simulink model "Robot"  (R2026a)
settings: Solver=ode1  StopTime=30  FixedStep=2e-5
model workspace (MAT data in the model file):
  bt_seed = 0
  pose0 = [0; 0; 0]
  theta_seed = 0
  x_seed = 0
  y_seed = 0
values from neighbouring files (symbols this model uses):
  bias_th = 0.000    (= 0)    [run_simulation.m]
  bias_x = 0.000    (= 0)    [run_simulation.m]
  bias_y = 0.000    (= 0)    [run_simulation.m]
  CAM_LAT = 0.08    [run_simulation.m]
  L_track = 0.136    [run_simulation.m]
  R_wheel = 0.065/2    (= 0.0325)    [run_simulation.m]
  sig_th = 0.035    [run_simulation.m]
  sig_xy = 0.002    [run_simulation.m]
  Ts_cam = 1/25    (= 0.04)    [run_simulation.m]
settings Model: ParameterArgumentNames=bt_seed,pose0,theta_seed,x_seed,y_seed  Creator=AdrianStark  LastModifiedBy=AdrianStark
settings ModelReferenceCC: ModelReferenceMinAlgLoopOccurrences=on

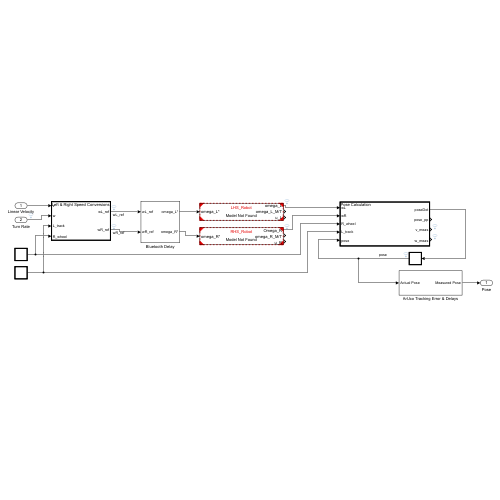
[thumbnail: Simulink's stored preview of the top-level diagram]
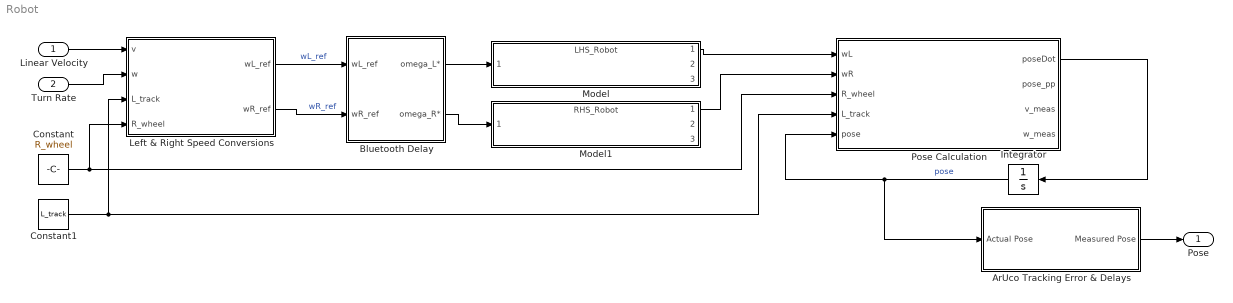
== system Robot ==
  Linear Velocity : Inport
  Turn Rate : Inport  Port=2
  ArUco Tracking Error & Delays : Subsystem
  Bluetooth Delay : Subsystem
  Constant : Constant  Value=R_wheel
  Constant1 : Constant  Value=L_track
  Integrator : Integrator  InitialCondition=pose0
  Left & Right Speed Conversions : MATLAB Function  TreatAsAtomicUnit=on
  Model : ModelReference  ModelNameDialog=LHS_Robot  SimulationMode=Normal  ModelReferenceVersion=1.40
  Model1 : ModelReference  ModelNameDialog=RHS_Robot  SimulationMode=Normal  ModelReferenceVersion=1.40
  Pose Calculation : MATLAB Function  TreatAsAtomicUnit=on
  Pose : Outport
  wires:
  Linear Velocity/1 -> Left & Right Speed Conversions/1(v)
  Turn Rate/1 -> Left & Right Speed Conversions/2(w)
  Pose Calculation/1(poseDot) -> Integrator/1
  Integrator/1 -> ArUco Tracking Error & Delays/1(Actual Pose), Pose Calculation/5(pose)  "pose"
  Constant/1 -> Left & Right Speed Conversions/4(R_wheel), Pose Calculation/3(R_wheel)
  Constant1/1 -> Left & Right Speed Conversions/3(L_track), Pose Calculation/4(L_track)
  Bluetooth Delay/1(omega_L*) -> Model/1
  Bluetooth Delay/2(omega_R*) -> Model1/1
  Left & Right Speed Conversions/2(wR_ref) -> Bluetooth Delay/2(wR_ref)  "wR_ref"
  Left & Right Speed Conversions/1(wL_ref) -> Bluetooth Delay/1(wL_ref)  "wL_ref"
  ArUco Tracking Error & Delays/1(Measured Pose) -> Pose/1
  Model1/1 -> Pose Calculation/2(wR)
  Model/1 -> Pose Calculation/1(wL)

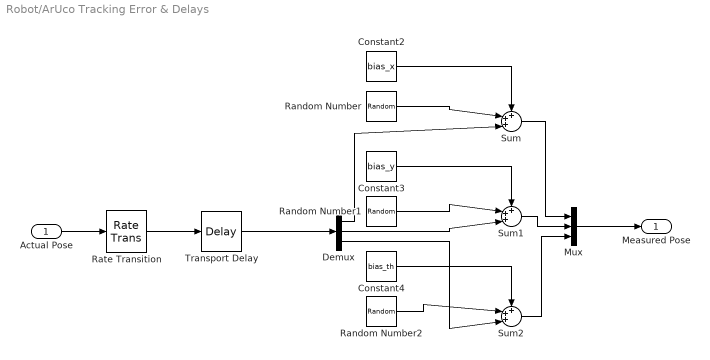
== system Robot/ArUco Tracking Error & Delays ==
  Actual Pose : Inport
  Constant2 : Constant  Value=bias_x
  Constant3 : Constant  Value=bias_y
  Constant4 : Constant  Value=bias_th
  Demux : Demux  Outputs=3
  Mux : Mux  Inputs=3
  Random Number : RandomNumber  Variance=sig_xy^2  Seed=x_seed  SampleTime=Ts_cam
  Random Number1 : RandomNumber  Variance=sig_xy^2  Seed=y_seed  SampleTime=Ts_cam
  Random Number2 : RandomNumber  Variance=sig_th^2  Seed=theta_seed  SampleTime=Ts_cam
  Rate Transition : RateTransition  OutPortSampleTime=Ts_cam
  Sum : Sum  Inputs=+++|
  Sum1 : Sum  Inputs=+++|
  Sum2 : Sum  Inputs=+++|
  Transport Delay : TransportDelay  DelayTime=CAM_LAT  InitialOutput=pose0
  Measured Pose : Outport
  wires:
  Demux/2 -> Sum1/3
  Demux/3 -> Sum2/3
  Random Number/1 -> Sum/2
  Random Number1/1 -> Sum1/2
  Actual Pose/1 -> Rate Transition/1
  Rate Transition/1 -> Transport Delay/1
  Sum1/1 -> Mux/2
  Transport Delay/1 -> Demux/1
  Sum/1 -> Mux/1
  Sum2/1 -> Mux/3
  Constant3/1 -> Sum1/1
  Constant4/1 -> Sum2/1
  Random Number2/1 -> Sum2/2
  Constant2/1 -> Sum/1
  Demux/1 -> Sum/3
  Mux/1 -> Measured Pose/1

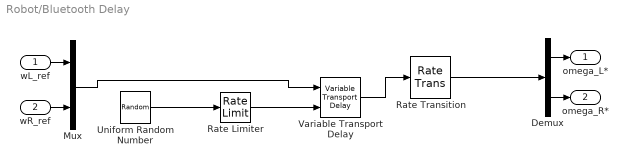
== system Robot/Bluetooth Delay ==
  wL_ref : Inport
  wR_ref : Inport  Port=2
  Demux : Demux  Outputs=2
  Mux : Mux  Inputs=2
  Rate Limiter : RateLimiter  RisingSlewLimit=0.8  FallingSlewLimit=-0.8  SampleTimeMode=inherited
  Rate Transition : RateTransition  Deterministic=off  OutPortSampleTime=Ts
  Uniform Random Number : UniformRandomNumber  Minimum=0.139  Maximum=0.268  Seed=bt_seed  SampleTime=0.1
  Variable Transport Delay : VariableTransportDelay  VariableDelayType=Variable transport delay  MaximumDelay=0.4  MaximumPoints=15000
  omega_L* : Outport
  omega_R* : Outport  Port=2
  wires:
  Variable Transport Delay/1 -> Rate Transition/1
  Demux/2 -> omega_R*/1
  Uniform Random Number/1 -> Rate Limiter/1
  wL_ref/1 -> Mux/1
  wR_ref/1 -> Mux/2
  Rate Transition/1 -> Demux/1
  Rate Limiter/1 -> Variable Transport Delay/2
  Mux/1 -> Variable Transport Delay/1
  Demux/1 -> omega_L*/1

== matlab function Robot/Pose Calculation ==
  data: wL input; poseDot output; wR input; pose_pp output; v_meas output; w_meas output; R_wheel input; L_track input; pose input
function [poseDot, pose_pp, v_meas, w_meas] = diffDriveOdometry(wL, wR, R_wheel, L_track, pose)

theta = pose(3);

v_meas = R_wheel*(wR + wL)/2;
w_meas = R_wheel*(wR - wL)/L_track;

poseDot = [ v_meas*cos(theta); ...
            v_meas*sin(theta); ...
            w_meas ];

thWrapped = theta - 2*pi*floor((theta + pi)/(2*pi));
pose_pp = [pose(1); pose(2); thWrapped];
end

== matlab function Robot/Left & Right Speed Conversions ==
  data: v input; wL_ref output; w input; wR_ref output; L_track input; R_wheel input
function [wL_ref, wR_ref] = diffDriveInverse(v, w, L_track, R_wheel)
wL_ref = (v - w*L_track/2) / R_wheel;
wR_ref = (v + w*L_track/2) / R_wheel;

%wL_ref = min(max(wL_ref, 0), W_MAX);
%wR_ref = min(max(wR_ref, 0), W_MAX);
end
